simulink model "Low_High_Filter"  (R2024a)
settings: Solver=FixedStepAuto  StartTime=0.0  StopTime=10  FixedStep=0.001  RelTol=1e-3
settings Model: Creator=Sanagostar  LastModifiedBy=Sanagostar

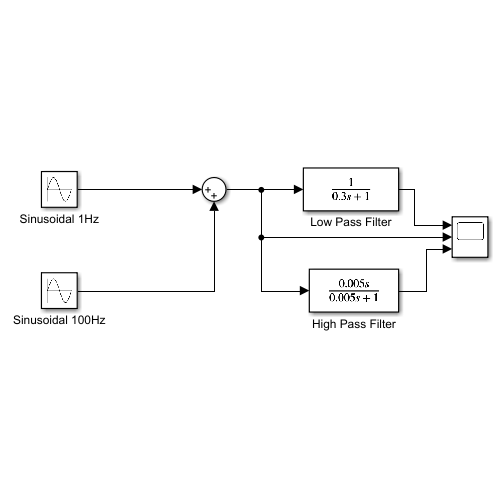
[thumbnail: Simulink's stored preview of the top-level diagram]
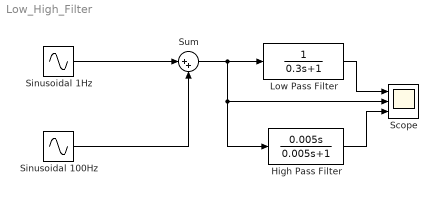
== system Low_High_Filter ==
  High Pass Filter : TransferFcn  Numerator=[0.005 0]  Denominator=[0.005 1]
  Low Pass Filter : TransferFcn  Denominator=[0.3 1]
  Scope : Scope  NumInputPorts=3
  Sinusoidal 100Hz : Sin  Frequency=100  SampleTime=0
  Sinusoidal 1Hz : Sin  Amplitude=5  SampleTime=0
  Sum : Sum  Inputs=|++
  wires:
  Sinusoidal 1Hz/1 -> Sum/1
  Sinusoidal 100Hz/1 -> Sum/2
  Sum/1 -> High Pass Filter/1, Scope/2, Low Pass Filter/1
  Low Pass Filter/1 -> Scope/1
  High Pass Filter/1 -> Scope/3
